simulink model "force_position_step3"  (R2025b)
settings: Solver=VariableStepAuto  StartTime=0.0  StopTime=2  RelTol=1e-3
values from neighbouring files (symbols this model uses):
  lut_i_mA = interp1(z_anchor_um, i_anchor_mA, lut_z_um, 'pchip')    [init_force_position_sim_step2.m]
  lut_z_um = linspace(min(z_anchor_um), max(z_anchor_um), 501)    [init_force_position_sim_step2.m]
settings Model: Creator=HYB  LastModifiedBy=HYB

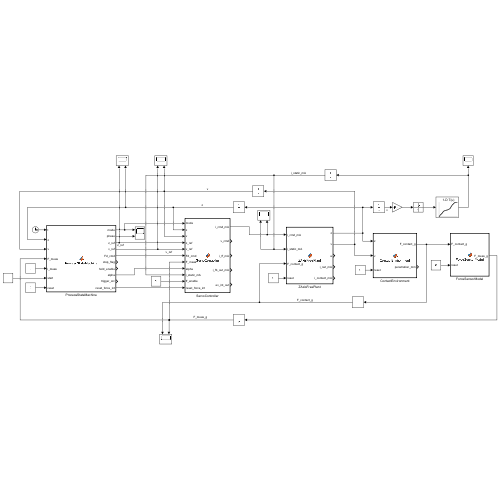
[thumbnail: Simulink's stored preview of the top-level diagram]
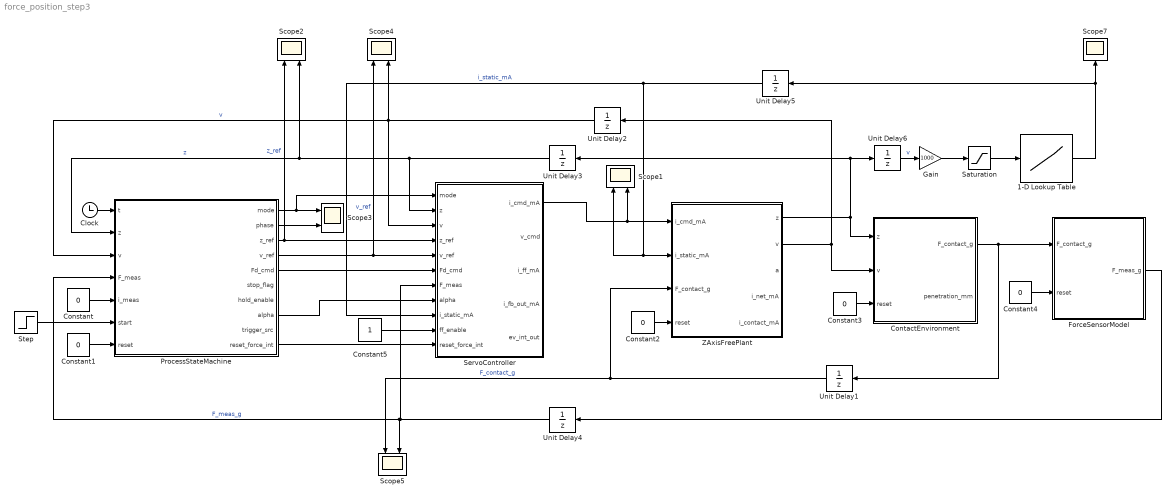
== system force_position_step3 ==
  1-D Lookup Table : Lookup_n-D  NumberOfTableDimensions=1  BreakpointsForDimension1=lut_z_um  Table=lut_i_mA  InternalRulePriority=Speed  RndMeth=Simplest
  Clock : Clock
  Constant{,1..4} (5 alike) : Constant  Value=0
  Constant5 : Constant
  ContactEnvironment : MATLAB Function  TreatAsAtomicUnit=on
  ForceSensorModel : MATLAB Function  TreatAsAtomicUnit=on
  Gain : Gain  Gain=1000
  ProcessStateMachine : MATLAB Function  TreatAsAtomicUnit=on
  Saturation : Saturate  UpperLimit=15000  LowerLimit=0
  Scope{1..5} (5 alike) : Scope  NumInputPorts=2
      Scope1 settings: ActiveDisplayYMinimum=-2033.0312996821785  ActiveDisplayYMaximum=2935.5773166551185
      Scope2 settings: ActiveDisplayYMinimum=14.137400388551367  ActiveDisplayYMaximum=14.510583605478384
      Scope3 settings: ActiveDisplayYMinimum=-0.49999999999999989  ActiveDisplayYMaximum=4.5  DataLoggingVariableName=ScopeData3
      Scope4 settings: ActiveDisplayYMinimum=-1.2472676873549906  ActiveDisplayYMaximum=0.58518359311440049  DataLoggingVariableName=ScopeData2
      Scope5 settings: ActiveDisplayYMinimum=-31.200728720443287  ActiveDisplayYMaximum=44.230982230865287  DataLoggingVariableName=ScopeData4
  Scope7 : Scope
      settings: ActiveDisplayYMinimum=645.6688347730925  ActiveDisplayYMaximum=873.33389076398271  DataLoggingVariableName=ScopeData7
  ServoController : MATLAB Function  TreatAsAtomicUnit=on
  Step : Step  Time=0.01  SampleTime=0
  Unit Delay{1..6} (6 alike) : UnitDelay  SampleTime=0.001  HasFrameUpgradeWarning=on
  ZAxisFreePlant : MATLAB Function  TreatAsAtomicUnit=on
  wires:
  ProcessStateMachine/1(mode) -> Scope3/1, ServoController/1(mode)
  ProcessStateMachine/3(z_ref) -> ServoController/4(z_ref), Scope2/1  "z_ref"
  ProcessStateMachine/4(v_ref) -> Scope4/1, ServoController/5(v_ref)  "v_ref"
  ProcessStateMachine/5(Fd_cmd) -> ServoController/6(Fd_cmd)
  ProcessStateMachine/10(reset_force_int) -> ServoController/11(reset_force_int)
  ProcessStateMachine/8(alpha) -> ServoController/8(alpha)
  ServoController/1(i_cmd_mA) -> Scope1/2, ZAxisFreePlant/1(i_cmd_mA)
  ZAxisFreePlant/1(z) -> ContactEnvironment/1(z), Unit Delay6/1, Unit Delay3/1
  ContactEnvironment/1(F_contact_g) -> ForceSensorModel/1(F_contact_g), Unit Delay1/1
  ForceSensorModel/1(F_meas_g) -> Unit Delay4/1
  Unit Delay4/1 -> Scope5/2, ProcessStateMachine/4(F_meas), ServoController/7(F_meas)  "F_meas_g"
  Unit Delay1/1 -> Scope5/1, ZAxisFreePlant/3(F_contact_g)  "F_contact_g"
  ZAxisFreePlant/2(v) -> ContactEnvironment/2(v), Unit Delay2/1
  Clock/1 -> ProcessStateMachine/1(t)
  Constant/1 -> ProcessStateMachine/5(i_meas)
  Step/1 -> ProcessStateMachine/6(start)
  Constant1/1 -> ProcessStateMachine/7(reset)
  Constant2/1 -> ZAxisFreePlant/4(reset)
  Constant3/1 -> ContactEnvironment/3(reset)
  Constant4/1 -> ForceSensorModel/2(reset)
  Unit Delay2/1 -> ProcessStateMachine/3(v), Scope4/2, ServoController/3(v)  "v"
  Unit Delay3/1 -> ServoController/2(z), Scope2/2, ProcessStateMachine/2(z)  "z"
  Saturation/1 -> 1-D Lookup Table/1
  Gain/1 -> Saturation/1
  1-D Lookup Table/1 -> Scope7/1, Unit Delay5/1
  Unit Delay5/1 -> ZAxisFreePlant/2(i_static_mA), Scope1/1, ServoController/9(i_static_mA)  "i_static_mA"
  Constant5/1 -> ServoController/10(ff_enable)
  ProcessStateMachine/2(phase) -> Scope3/2
  Unit Delay6/1 -> Gain/1  "v"

== matlab function force_position_step3/ForceSensorModel ==
  data: F_contact_g input; F_meas_g output; reset input
function F_meas_g = ForceSensorModel(F_contact_g, reset)
%#codegen

% ============================================================
% 力传感器模型：一阶低通 + 离散延迟
% 输入：真实接触力 F_contact_g
% 输出：测得力 F_meas_g
% ============================================================

%% 参数
Ts = 1e-3;          % 1 ms
tau_s = 0.003;      % 传感器/滤波时间常数，3 ms
delay_steps = 1;    % 传感器延迟，1个采样周期，即1 ms

alpha = Ts / (tau_s + Ts);

persistent F_filt delay_buf

if isempty(F_filt)
    F_filt = 0.0;
    delay_buf = zeros(1, delay_steps + 1);
end

if reset
    F_filt = 0.0;
    delay_buf = zeros(1, delay_steps + 1);
end

%% 一阶低通滤波
F_filt = F_filt + alpha * (F_contact_g - F_filt);

%% 离散延迟
F_meas_g = delay_buf(delay_steps + 1);

for k = delay_steps + 1:-1:2
    delay_buf(k) = delay_buf(k-1);
end

delay_buf(1) = F_filt;

== matlab function force_position_step3/ContactEnvironment ==
  data: z input; F_contact_g output; v input; reset input; penetration_mm output
function [F_contact_g, penetration_mm] = ContactEnvironment(z, v, reset)
%#codegen

% ============================================================
% 接触环境模型：Kelvin-Voigt 接触模型
% z: mm，下压为正
% v: mm/s，下压为正
% ============================================================

z_contact = 14.30;        % 接触位置，mm
Ke_g_per_mm = 800.0;      % 接触刚度，g/mm
Be_g_per_mms = 50.0;      % 接触阻尼，g/(mm/s)

penetration_mm = z - z_contact;

if penetration_mm < 0.0
    penetration_mm = 0.0;
end

if penetration_mm > 0.0
    F_contact_g = Ke_g_per_mm * penetration_mm + Be_g_per_mms * v;
else
    F_contact_g = 0.0;
end

% 不允许拉力
if F_contact_g < 0.0
    F_contact_g = 0.0;
end

== matlab function force_position_step3/ZAxisFreePlant ==
  data: i_cmd_mA input; z output; i_static_mA input; F_contact_g input; reset input; v output; a output; i_net_mA output; i_contact_mA output
function [z, v, a, i_net_mA, i_contact_mA] = ZAxisFreePlant(i_cmd_mA, i_static_mA, F_contact_g, reset)
%#codegen

% ============================================================
% Z轴对象模型：自由运动 + 静态非线性负载 + 接触反作用力
% 下行方向为正
% z: mm
% v: mm/s
% 电流: mA
% F_contact_g: 真实接触力，g
% ============================================================

%% 参数
Ts = 1e-3;

z0 = 0.0;
v0 = 0.0;

z_min = 0.0;
z_max = 15.2;

Kacc = 20.0;          % mm/s^2 per mA
Cv_mA = 1.0;          % mA/(mm/s)
Icoul_mA = 2.0;       % mA
vs = 0.05;            % mm/s

v_limit = 200.0;      % mm/s，仿真保护

% 接触力到等效反作用电流
Kcontact_mA_per_g = 1.0;    % mA/g，初版取1，后续可标定

persistent z_k v_k

if isempty(z_k)
    z_k = z0;
    v_k = v0;
end

if reset
    z_k = z0;
    v_k = v0;
end

%% 摩擦电流
i_fric_mA = Cv_mA * v_k + Icoul_mA * tanh(v_k / vs);

%% 接触反作用电流
i_contact_mA = Kcontact_mA_per_g * F_contact_g;

%% 净驱动电流
i_net_mA = i_cmd_mA - i_static_mA - i_fric_mA - i_contact_mA;

%% 加速度
a = Kacc * i_net_mA;

%% 积分
v_k = v_k + Ts * a;

%% 速度限幅
if v_k > v_limit
    v_k = v_limit;
elseif v_k < -v_limit
    v_k = -v_limit;
end

z_k = z_k + Ts * v_k;

%% 行程限位
if z_k < z_min
    z_k = z_min;
    if v_k < 0
        v_k = 0.0;
    end
elseif z_k > z_max
    z_k = z_max;
    if v_k > 0
        v_k = 0.0;
    end
end

z = z_k;
v = v_k;

== matlab function force_position_step3/ServoController ==
  data: mode input; i_cmd_mA output; z input; v input; z_ref input; v_ref input; Fd_cmd input; F_meas input; alpha input; i_static_mA input; ff_enable input; reset_force_int input; v_cmd output; i_ff_mA output; i_fb_out_mA output; ev_int_out output
function [i_cmd_mA, v_cmd, i_ff_mA, i_fb_out_mA, ev_int_out] = ServoController( ...
    mode, z, v, z_ref, v_ref, Fd_cmd, F_meas, alpha, ...
    i_static_mA, ff_enable, reset_force_int)
%#codegen

% ============================================================
% 简化伺服控制器：
% mode = 1: 位置模式，位置外环生成速度指令，速度PI输出电流
% mode = 2: 速度模式，速度PI输出电流
% mode = 3: 接触后力矩/前馈保压模式
%           当前阶段采用：
%           静态前馈 + 温和速度阻尼 + 速度门控力前馈
%           先关闭力闭环反馈
% mode = 9: 安全停止
% ============================================================

%% 基本参数
Ts = 1e-3;

%% 位置环参数
Kp_pos = 100.0;
v_fast_max = 100.0;

%% 速度PI参数，mode 1/2 使用
Kvp = 20.0;
Kvi = 200.0;

i_limit = 5000.0;
i_v_int_limit = 3000.0;

%% 力前馈参数
% 第一步排查时先设为0
% 等稳定后再改为 0.2, 0.3, 0.5
Kff_force_mA_per_g = 0.2;

%% 力反馈参数
% 当前阶段先关闭力闭环反馈
Kpf = 0.0;
Kif = 0.0;
i_force_int_limit = 500.0;

%% mode=3 接触缓冲与前馈门控参数
T_brake = 0.020;        % 进入mode=3后至少先缓冲20ms
v_hold_th = 0.3;        % 速度小于该值才允许增加力前馈，mm/s

T_ramp_ff = 0.120;      % 力前馈引入时间，先慢一点
T_release = 0.020;      % 速度过大时 alpha_ff 退回时间

% 关键修改：阻尼不要太大
Kd_brake = 10.0;        % 接触缓冲阶段速度阻尼，mA/(mm/s)
Kd_hold  = 5.0;         % 准静态前馈阶段速度阻尼，mA/(mm/s)

% 关键修改：阻尼电流限幅
i_damp_limit = 300.0;   % mA

% 关键修改：小速度死区，避免小速度附近抖动
v_damp_deadband = 0.05; % mm/s

%% 持久变量
persistent ev_int eF_int last_mode alpha_ff hold_timer

if isempty(ev_int)
    ev_int = 0.0;
    eF_int = 0.0;
    last_mode = 0.0;
    alpha_ff = 0.0;
    hold_timer = 0.0;
end

%% 默认输出和内部变量
v_cmd = 0.0;

i_speed_fb_mA = 0.0;
i_force_ff_mA = 0.0;
i_force_fb_mA = 0.0;
i_damp_mA = 0.0;

e_v = 0.0;
eF = 0.0;

%% 进入 mode=3 瞬间清理运动阶段残留
if last_mode ~= 3.0 && mode == 3.0
    ev_int = 0.0;
    eF_int = 0.0;
    alpha_ff = 0.0;
    hold_timer = 0.0;
end

%% 外部复位力控积分
if reset_force_int
    eF_int = 0.0;
end

%% 安全停止时清空积分
if mode == 9.0
    ev_int = 0.0;
    eF_int = 0.0;
    alpha_ff = 0.0;
    hold_timer = 0.0;
end

%% 静态前馈
if ff_enable > 0.5
    i_ff_mA = i_static_mA;
else
    i_ff_mA = 0.0;
end

%% ============================================================
%  mode 1：位置模式
% ============================================================
if mode == 1.0

    e_pos = z_ref - z;
    v_cmd = Kp_pos * e_pos;

    if v_cmd > v_fast_max
        v_cmd = v_fast_max;
    elseif v_cmd < -v_fast_max
        v_cmd = -v_fast_max;
    end

    e_v = v_cmd - v;
    i_p = Kvp * e_v;

    ev_int = ev_int + e_v * Ts;
    i_i = Kvi * ev_int;

    if i_i > i_v_int_limit
        i_i = i_v_int_limit;
        ev_int = i_i / Kvi;
    elseif i_i < -i_v_int_limit
        i_i = -i_v_int_limit;
        ev_int = i_i / Kvi;
    end

    i_speed_fb_mA = i_p + i_i;

%% ============================================================
%  mode 2：速度模式
% ============================================================
elseif mode == 2.0

    v_cmd = v_ref;

    e_v = v_cmd - v;
    i_p = Kvp * e_v;

    ev_int = ev_int + e_v * Ts;
    i_i = Kvi * ev_int;

    if i_i > i_v_int_limit
        i_i = i_v_int_limit;
        ev_int = i_i / Kvi;
    elseif i_i < -i_v_int_limit
        i_i = -i_v_int_limit;
        ev_int = i_i / Kvi;
    end

    i_speed_fb_mA = i_p + i_i;

%% ============================================================
%  mode 3：接触后前馈/阻尼模式
% ============================================================
elseif mode == 3.0

    v_cmd = 0.0;
    i_speed_fb_mA = 0.0;

    hold_timer = hold_timer + Ts;

    %% 1. 判断当前是否处于缓冲阶段
    if (hold_timer < T_brake) || (abs(v) > v_hold_th)

        % 缓冲阶段：不引入力前馈，只做速度阻尼
        Kd_now = Kd_brake;

        % 速度过大时，alpha_ff 不增加，甚至退回
        alpha_ff = alpha_ff - Ts / T_release;

        if alpha_ff < 0.0
            alpha_ff = 0.0;
        elseif alpha_ff > 1.0
            alpha_ff = 1.0;
        end

        i_force_ff_mA = 0.0;
        i_force_fb_mA = 0.0;

    else

        % 准静态阶段：速度足够小，允许缓慢引入力前馈
        Kd_now = Kd_hold;

        alpha_ff = alpha_ff + Ts / T_ramp_ff;

        if alpha_ff > 1.0
            alpha_ff = 1.0;
        elseif alpha_ff < 0.0
            alpha_ff = 0.0;
        end

        % 外部 alpha 和内部 alpha_ff 取较小值
        if alpha < alpha_ff
            alpha_ff_eff = alpha;
        else
            alpha_ff_eff = alpha_ff;
        end

        i_force_ff_mA = alpha_ff_eff * Kff_force_mA_per_g * Fd_cmd;

        % 当前先关闭力闭环反馈
        eF = Fd_cmd - F_meas;

        if Kpf > 0.0 || Kif > 0.0

            if Kif > 0.0
                eF_int = eF_int + eF * Ts;
                i_force_i = Kif * eF_int;

                if i_force_i > i_force_int_limit
                    i_force_i = i_force_int_limit;
                    eF_int = i_force_i / Kif;
                elseif i_force_i < -i_force_int_limit
                    i_force_i = -i_force_int_limit;
                    eF_int = i_force_i / Kif;
                end
            else
                i_force_i = 0.0;
                eF_int = 0.0;
            end

            i_force_fb_mA = Kpf * eF + i_force_i;

        else
            i_force_fb_mA = 0.0;
            eF_int = 0.0;
        end
    end

    %% 2. 速度阻尼项
    if abs(v) < v_damp_deadband
        i_damp_mA = 0.0;
    else
        i_damp_mA = -Kd_now * v;
    end

    %% 3. 阻尼电流限幅
    if i_damp_mA > i_damp_limit
        i_damp_mA = i_damp_limit;
    elseif i_damp_mA < -i_damp_limit
        i_damp_mA = -i_damp_limit;
    end

%% ============================================================
%  mode 9：安全停止
% ============================================================
elseif mode == 9.0

    v_cmd = 0.0;
    i_ff_mA = 0.0;
    i_speed_fb_mA = 0.0;
    i_force_ff_mA = 0.0;
    i_force_fb_mA = 0.0;
    i_damp_mA = 0.0;

else

    v_cmd = 0.0;
    i_speed_fb_mA = 0.0;
    i_force_ff_mA = 0.0;
    i_force_fb_mA = 0.0;
    i_damp_mA = 0.0;

end

%% 合成未限幅电流
i_cmd_unsat = i_ff_mA + i_speed_fb_mA + i_force_ff_mA + i_force_fb_mA + i_damp_mA;

%% 总电流限幅
i_cmd_mA = i_cmd_unsat;

if i_cmd_mA > i_limit
    i_cmd_mA = i_limit;
elseif i_cmd_mA < -i_limit
    i_cmd_mA = -i_limit;
end

%% 速度模式抗积分饱和
if (mode == 1.0 || mode == 2.0)
    if i_cmd_unsat ~= i_cmd_mA
        if (i_cmd_unsat > i_limit && e_v > 0.0) || (i_cmd_unsat < -i_limit && e_v < 0.0)
            ev_int = ev_int - 0.5 * e_v * Ts;
        end
    end
end

%% 力控模式抗积分饱和
if mode == 3.0
    if i_cmd_unsat ~= i_cmd_mA
        if (i_cmd_unsat > i_limit && eF > 0.0) || (i_cmd_unsat < -i_limit && eF < 0.0)
            eF_int = eF_int - 0.5 * eF * Ts;
        end
    end
end

%% 输出观测量
if mode == 3.0
    i_fb_out_mA = i_force_fb_mA;
else
    i_fb_out_mA = i_speed_fb_mA;
end

% 默认输出速度积分
% 调试 alpha_ff 时，可以临时改成：ev_int_out = alpha_ff;
ev_int_out = ev_int;

last_mode = mode;

== matlab function force_position_step3/ProcessStateMachine ==
  data: t input; mode output; z input; v input; F_meas input; i_meas input; start input; reset input; phase output; z_ref output; v_ref output; Fd_cmd output; stop_flag output; hold_enable output; alpha output; trigger_src output; reset_force_int output
function [mode, phase, z_ref, v_ref, Fd_cmd, stop_flag, hold_enable, alpha, trigger_src, reset_force_int] = ...
    ProcessStateMachine(t, z, v, F_meas, i_meas, start, reset)
%#codegen

% ============================================================
% 力位控制工艺流程状态机
% 阶段：
% 0 Ready
% 1 FastPosition: 位置模式快进到 13 mm
% 2 FirstVelocity: 第一速度到 14 mm
% 3 SearchVelocity: 第二速度搜索接触
% 4 ForceHold: 力矩/电流模式保压
% 5 ErrorStop: 超行程或异常停止
% ============================================================


%% ---------- 可调参数 ----------
z_fast_end = 13.0;     % mm
z_v1_end   = 14.0;     % mm
z_max      = 15.0;     % mm

pos_tol = 0.02;        % mm

v1_search = 10.0;       % mm/s
v2_search = 2.0;       % mm/s

F_th = 10.0;           % g
T_force_confirm = 0.001;   % s

v_stop_th = 0.05;          % mm/s
T_v_confirm = 0.005;       % s

% 第一版暂不启用电流判断，所以阈值给很大
i_stop_th = 1e9;
T_i_confirm = 0.003;       % s

Fd_set = 200.0;            % g
T_ramp_force = 0.010;      % s

%% ---------- 状态变量 ----------
persistent state t_enter tF_start tV_start tI_start prev_state

if isempty(state)
    state = int32(0);
    prev_state = int32(0);
    t_enter = 0.0;
    tF_start = -1.0;
    tV_start = -1.0;
    tI_start = -1.0;
end

if reset
    state = int32(0);
    prev_state = int32(0);
    t_enter = t;
    tF_start = -1.0;
    tV_start = -1.0;
    tI_start = -1.0;
end

%% ---------- 默认输出 ----------
mode = 0;
phase = double(state);
z_ref = z; % 默认保持住位置，防止突然运动
v_ref = 0.0;
Fd_cmd = Fd_set; % 默认力指令就设置为力设定值，切换为力控时目标力则已经是设定值
stop_flag = false; % 默认不停止，运行外部控制器继续执行位置/速度环
hold_enable = false; % 默认禁用积分器保持，在状态4会开启，力控时造成的位移累积误差在切换回位控时可以快速恢复
alpha = 0.0; % 在状态4时会从0平滑过渡到1
trigger_src = 0;       % 0 none, 1 force, 2 velocity, 3 current, 4 z_max
reset_force_int = false; % 默认不复位力控积分器，只在进入状态4的瞬间设1

prev_state = state;

%% ---------- 启动逻辑 ----------
if state == 0
    mode = 0;
    phase = 0;
    z_ref = z;
    v_ref = 0.0;
    alpha = 0.0;
    
    if start % 一般阶跃输入
        state = int32(1);
        t_enter = t; % 进入当前状态的时间戳
    end
end

%% ---------- 状态 1：位置快进 ----------
if state == 1
    mode = 1;
    phase = 1;
    z_ref = z_fast_end;
    v_ref = 0.0;
    alpha = 0.0;
    
    if z >= z_fast_end - pos_tol
        state = int32(2);
        t_enter = t;
    end
end

%% ---------- 状态 2：第一速度 ----------
if state == 2
    mode = 2;          % 速度模式
    phase = 2;
    z_ref = z;
    v_ref = v1_search;
    alpha = 0.0;
    
    if z >= z_v1_end - pos_tol
        state = int32(3);
        t_enter = t;
        tF_start = -1.0;
        tV_start = -1.0;
        tI_start = -1.0;
    end
end

%% ---------- 状态 3：第二速度搜索 ----------
if state == 3
    mode = 2;          % 速度模式
    phase = 3;
    z_ref = z;
    v_ref = v2_search;
    alpha = 0.0;
    
    % --- 压力触发 ---
    if F_meas > F_th
        if tF_start < 0.0
            tF_start = t;
        end
    else
        tF_start = -1.0;
    end
    
    force_ok = false;
    if tF_start >= 0.0
        if (t - tF_start) >= T_force_confirm
            force_ok = true;
        end
    end
    
    % --- 速度触发，第一版作为备用 ---
    if abs(v) < v_stop_th
        if tV_start < 0.0
            tV_start = t;
        end
    else
        tV_start = -1.0;
    end
    
    velocity_ok = false;
    if tV_start >= 0.0
        if (t - tV_start) >= T_v_confirm
            velocity_ok = true;
        end
    end
    
    % --- 电流触发，第一版实际不会触发 ---
    if abs(i_meas) > i_stop_th
        if tI_start < 0.0
            tI_start = t;
        end
    else
        tI_start = -1.0;
    end
    
    current_ok = false;
    if tI_start >= 0.0
        if (t - tI_start) >= T_i_confirm
            current_ok = true;
        end
    end
    
    % --- 停止条件 ---
    if force_ok
        state = int32(4);
        t_enter = t;
        trigger_src = 1;
        stop_flag = true;
    elseif velocity_ok
        state = int32(4);
        t_enter = t;
        trigger_src = 2;
        stop_flag = true;
    elseif current_ok
        state = int32(4);
        t_enter = t;
        trigger_src = 3;
        stop_flag = true;
    elseif z >= z_max
        state = int32(5);
        t_enter = t;
        trigger_src = 4;
    end
end

%% ---------- 状态 4：力矩/电流模式保压 ----------
if state == 4
    mode = 3;          % 力矩/电流模式
    phase = 4;
    z_ref = z;
    v_ref = 0.0;
    Fd_cmd = Fd_set;
    stop_flag = true;
    hold_enable = true;
    
    % 目标力前馈平滑引入系数 alpha: 0 -> 1
    tau = (t - t_enter) / T_ramp_force;
    if tau < 0.0
        tau = 0.0;
    elseif tau > 1.0
        tau = 1.0;
    end
    
    % S型平滑
    alpha = 3.0*tau*tau - 2.0*tau*tau*tau;
end

%% ---------- 状态 5：安全停止 ----------
if state == 5
    mode = 9;
    phase = 5;
    z_ref = z;
    v_ref = 0.0;
    Fd_cmd = 0.0;
    stop_flag = true;
    hold_enable = false;
    alpha = 0.0;
end

%% ---------- 进入保压瞬间复位力控积分 ----------
if prev_state ~= int32(4) && state == int32(4)
    reset_force_int = true;
else
    reset_force_int = false;
end

phase = double(state);
